simulink model "UECM_1RC"  (R2026b)
settings: Solver=VariableStepAuto
model workspace (MAT data in the model file):
  C1 = nan
  C2 = nan
  R0 = nan
  R1 = nan
  R2 = nan
settings Model: Creator=chagyeongho  LastModifiedBy=chagyeongho

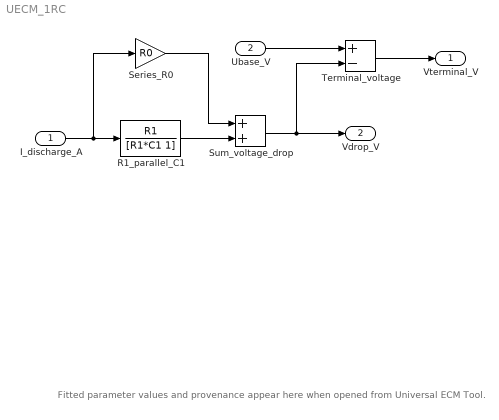
== system UECM_1RC ==
  note: Fitted parameter values and provenance appear here when opened from Universal ECM Tool.
  I_discharge_A : Inport  Interpolate=off
  Ubase_V : Inport  Port=2
  R1_parallel_C1 : TransferFcn  Numerator=R1  Denominator=[R1*C1 1]
  Series_R0 : Gain  Gain=R0
  Sum_voltage_drop : Sum
  Terminal_voltage : Sum  Inputs=+-
  Vterminal_V : Outport
  Vdrop_V : Outport  Port=2
  wires:
  Terminal_voltage/1 -> Vterminal_V/1
  Sum_voltage_drop/1 -> Terminal_voltage/2, Vdrop_V/1
  Ubase_V/1 -> Terminal_voltage/1
  R1_parallel_C1/1 -> Sum_voltage_drop/2
  Series_R0/1 -> Sum_voltage_drop/1
  I_discharge_A/1 -> Series_R0/1, R1_parallel_C1/1
